simulink model "hdlcordic_eml"  (R2026a)
settings: Solver=FixedStepDiscrete  StopTime=720
InitFcn:
  | rate = 8;
libraries: simulink_need_slupdate x2, simulink x1
Description:
  | CORDIC Algorithm Using the MATLAB(R) Function Block
  | This example shows how to use HDL Coder(TM) to check, generate and
  | verify HDL for a fixed-point CORDIC model implementing sin and cos
  | trigonometric functions using the MATLAB Function Block.
settings Model: Creator=The MathWorks, Inc.  LastModifiedBy=The MathWorks, Inc.
settings OptimizationCC: ConditionallyExecuteInputs=off  InitFltsAndDblsToZero=on  EfficientMapNaN2IntZero=off
settings DebuggingCC: SaveWithParameterizedLinksMsg=none  UnderspecifiedInitializationDetection=Classic  SingleTaskRateTransMsg=error  IntegerOverflowMsg=none  ParameterDowncastMsg=none  ParameterOverflowMsg=none  ParameterPrecisionLossMsg=none  ParameterTunabilityLossMsg=none  IntegerSaturationMsg=none
settings HardwareCC: ProdHWDeviceType=ASIC/FPGA  TargetHWDeviceType=32-bit Generic  ProdEqTarget=off
settings GRTTargetCC: TargetFcnLib=ansi_tfl_tmw_new.mat  CombineOutputUpdateFcns=off  GRTInterface=on

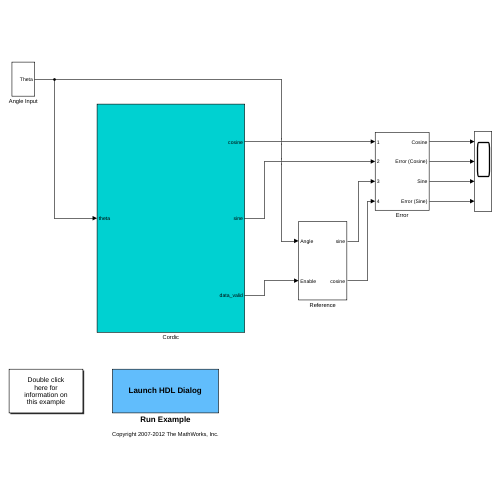
[thumbnail: Simulink's stored preview of the top-level diagram]
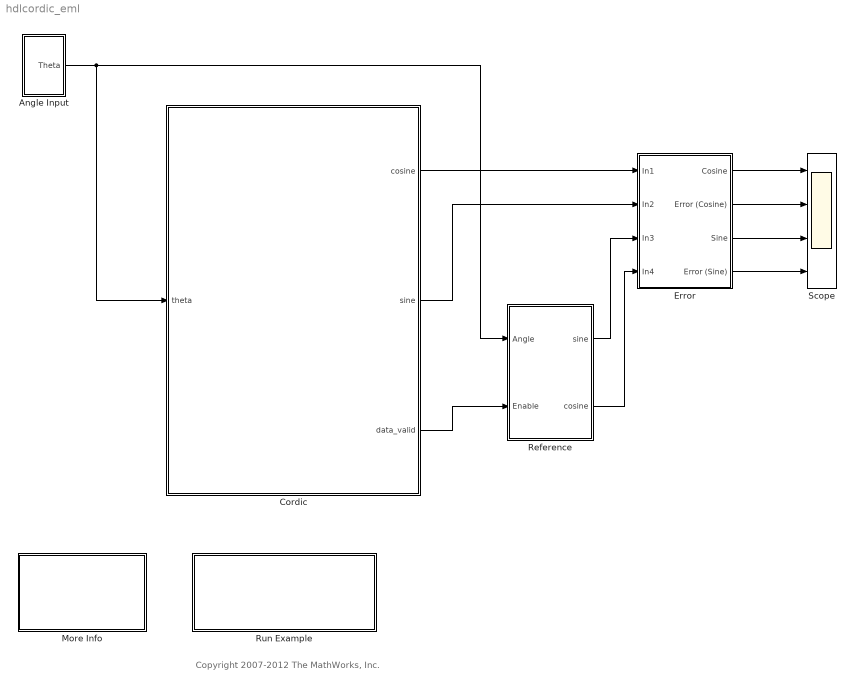
== system hdlcordic_eml ==
  note: Copyright 2007-2012 The MathWorks, Inc.
  Angle Input : Subsystem
  Cordic : Subsystem
  Error : Subsystem
  More Info : Subsystem
      mask Display: disp('Double click\nhere for\ninformation on\nthis example')
  Reference : Subsystem
  Run Example : Subsystem
      settings: OpenFcn=hdldialog(bdroot)
      mask Display: disp('Launch HDL Dialog')
  Scope : Scope  NumInputPorts=4
      settings: TimeSpan=800  Title=Cosine_Reference (Yellow) vs Cosine_Cordic (Purple)  ActiveDisplayYMinimum=-1  ActiveDisplayYMaximum=1
  wires:
  Angle Input/1(Theta) -> Reference/1(Angle), Cordic/1(theta)
  Reference/1(sine) -> Error/3(In3)
  Reference/2(cosine) -> Error/4(In4)
  Error/1(Cosine) -> Scope/1
  Error/2(Error (Cosine)) -> Scope/2
  Error/3(Sine) -> Scope/3
  Error/4(Error (Sine)) -> Scope/4
  Cordic/1(cosine) -> Error/1(In1)
  Cordic/2(sine) -> Error/2(In2)
  Cordic/3(data_valid) -> Reference/2(Enable)

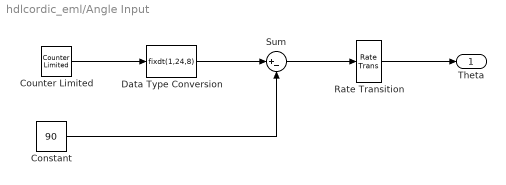
== system hdlcordic_eml/Angle Input ==
  Constant : Constant  Value=90  OutDataTypeStr=fixdt(1,24,8)  SampleTime=1
  Counter Limited : simulink/Sources/Counter Limited  uplimit=360  tsamp=1
  Data Type Conversion : DataTypeConversion  OutDataTypeStr=fixdt(1,24,8)  SaturateOnIntegerOverflow=off  RndMeth=Floor
  Rate Transition : RateTransition  OutPortSampleTime=1/rate
  Sum : Sum  Inputs=|+-  OutDataTypeStr=fixdt(1, 24, 8)
  Theta : Outport
  wires:
  Rate Transition/1 -> Theta/1
  Sum/1 -> Rate Transition/1
  Data Type Conversion/1 -> Sum/1
  Constant/1 -> Sum/2
  Counter Limited/1 -> Data Type Conversion/1

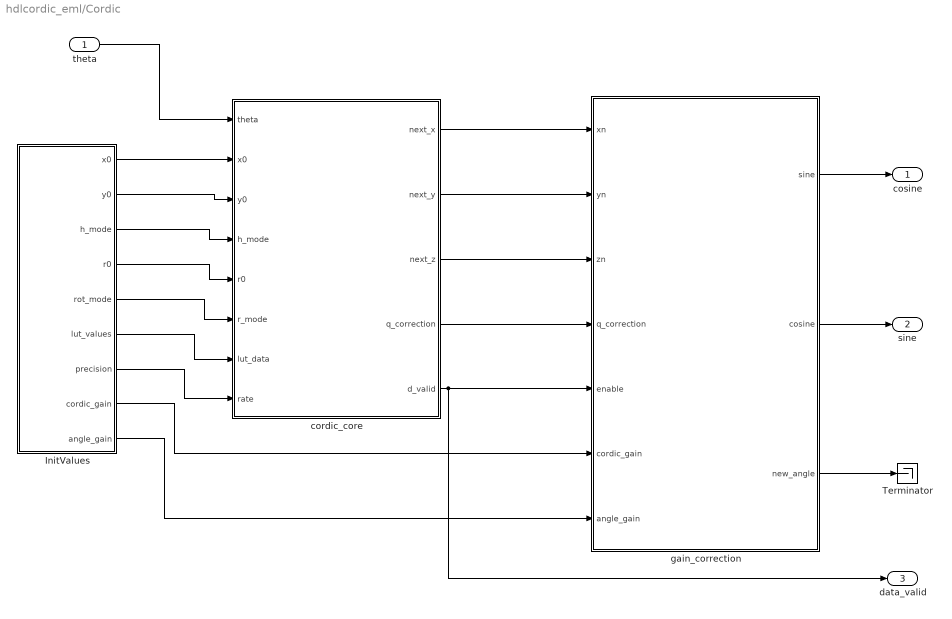
== system hdlcordic_eml/Cordic ==
  theta : Inport
  InitValues : Subsystem
  Terminator : Terminator
  cordic_core : Subsystem
  gain_correction : MATLAB Function  TreatAsAtomicUnit=on
  cosine : Outport
  sine : Outport  Port=2
  data_valid : Outport  Port=3
  wires:
  gain_correction/1(sine) -> cosine/1
  gain_correction/2(cosine) -> sine/1
  gain_correction/3(new_angle) -> Terminator/1
  cordic_core/1(next_x) -> gain_correction/1(xn)
  cordic_core/2(next_y) -> gain_correction/2(yn)
  cordic_core/3(next_z) -> gain_correction/3(zn)
  cordic_core/4(q_correction) -> gain_correction/4(q_correction)
  cordic_core/5(d_valid) -> gain_correction/5(enable), data_valid/1
  InitValues/8(cordic_gain) -> gain_correction/6(cordic_gain)
  InitValues/9(angle_gain) -> gain_correction/7(angle_gain)
  theta/1 -> cordic_core/1(theta)
  InitValues/1(x0) -> cordic_core/2(x0)
  InitValues/2(y0) -> cordic_core/3(y0)
  InitValues/3(h_mode) -> cordic_core/4(h_mode)
  InitValues/4(r0) -> cordic_core/5(r0)
  InitValues/5(rot_mode) -> cordic_core/6(r_mode)
  InitValues/6(lut_values) -> cordic_core/7(lut_data)
  InitValues/7(precision) -> cordic_core/8(rate)

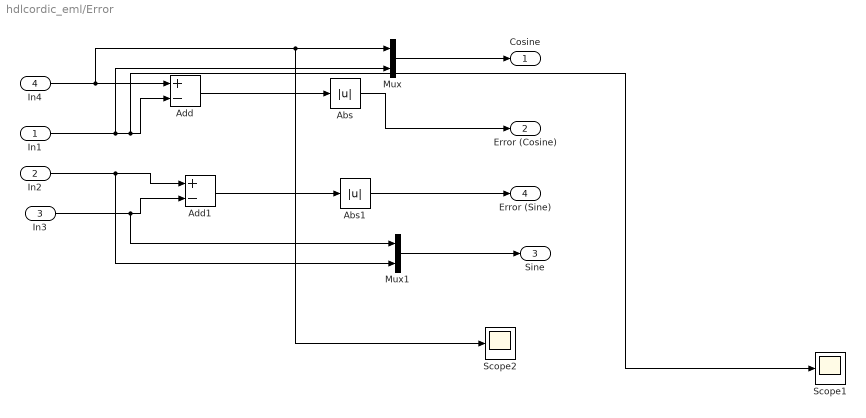
== system hdlcordic_eml/Error ==
  In1 : Inport
  In2 : Inport  Port=2
  In3 : Inport  Port=3
  In4 : Inport  Port=4
  Abs : Abs  SaturateOnIntegerOverflow=off
  Abs1 : Abs  SaturateOnIntegerOverflow=off
  Add : Sum  Inputs=+-  OutDataTypeStr=Inherit: Inherit via back propagation
  Add1 : Sum  Inputs=+-  OutDataTypeStr=Inherit: Inherit via back propagation
  Mux : Mux  Inputs=2
  Mux1 : Mux  Inputs=2
  Scope1 : Scope
      settings: ActiveDisplayYMinimum=0.7125  ActiveDisplayYMaximum=0.7875  DataLoggingVariableName=ScopeData3
  Scope2 : Scope
      settings: ActiveDisplayYMinimum=0.1  ActiveDisplayYMaximum=0.8  DataLoggingVariableName=ScopeData2
  Cosine : Outport
  Error (Cosine) : Outport  Port=2
  Sine : Outport  Port=3
  Error (Sine) : Outport  Port=4
  wires:
  In4/1 -> Add/1, Mux/1, Scope2/1
  In1/1 -> Mux/2, Add/2, Scope1/1
  In2/1 -> Add1/1, Mux1/2
  In3/1 -> Add1/2, Mux1/1
  Add1/1 -> Abs1/1
  Add/1 -> Abs/1
  Abs/1 -> Error (Cosine)/1
  Mux/1 -> Cosine/1
  Abs1/1 -> Error (Sine)/1
  Mux1/1 -> Sine/1

== system hdlcordic_eml/More Info ==
  note: MATLAB Function Block CORDIC Example
  note: This example shows how to implement the CORDIC algorithm solely using
      | MATLAB Function blocks.
      |
      | CORDIC is a shift-add based algorithm suitable for HDL code generation.
      | For complete details see the following reference paper.
      |
      | A survey of CORDIC algorithms for FPGAs
      | Ray Andraka, FPGA '98. Proceedings of the
      | 1998 ACM/SIGDA sixth international symposium on Field programmable gate arrays,
      | Feb. 22-24, 1998, Monterey, CA. pp191-200.
  note: For Verilog:
      |
      |   makehdl('hdlcordic_eml/Cordic', 'TargetLanguage', 'Verilog')
      |   makehdltb('hdlcordic_eml/Cordic', 'TargetLanguage', 'Verilog')
      |
      | For VHDL:
      |
      |   makehdl('hdlcordic_eml/Cordic', 'TargetLanguage', 'Vhdl')
      |   makehdltb('hdlcordic_eml/Cordic', 'TargetLanguage', 'Vhdl')
  note: In MATLAB(R), type the following:

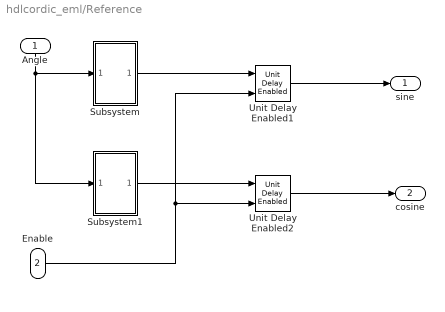
== system hdlcordic_eml/Reference ==
  Angle : Inport
  Enable : Inport  Port=2
  Subsystem : Subsystem
      mask Display: disp('Sine')
  Subsystem1 : Subsystem
      mask Display: disp('Cosine')
  Unit Delay Enabled1 : simulink_need_slupdate/Unit Delay Enabled  vinit=0  tsamp=1/rate
  Unit Delay Enabled2 : simulink_need_slupdate/Unit Delay Enabled  vinit=0  tsamp=1/rate
  sine : Outport
  cosine : Outport  Port=2
  wires:
  Angle/1 -> Subsystem/1(In1), Subsystem1/1(In1)
  Subsystem/1(Out1) -> Unit Delay Enabled1/1
  Unit Delay Enabled1/1 -> sine/1
  Enable/1 -> Unit Delay Enabled1/2, Unit Delay Enabled2/2
  Subsystem1/1(Out1) -> Unit Delay Enabled2/1
  Unit Delay Enabled2/1 -> cosine/1

== system hdlcordic_eml/Run Example ==

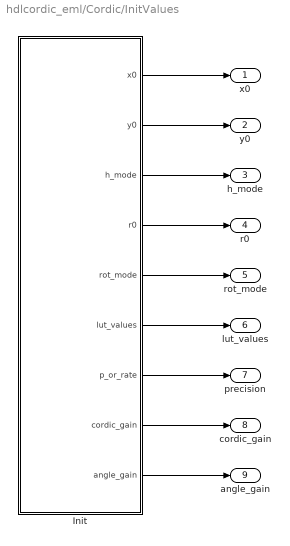
== system hdlcordic_eml/Cordic/InitValues ==
  Init : MATLAB Function  TreatAsAtomicUnit=on
  x0 : Outport
  y0 : Outport  Port=2
  h_mode : Outport  Port=3
  r0 : Outport  Port=4
  rot_mode : Outport  Port=5
  lut_values : Outport  Port=6
  precision : Outport  Port=7
  cordic_gain : Outport  Port=8
  angle_gain : Outport  Port=9
  wires:
  Init/1(x0) -> x0/1
  Init/2(y0) -> y0/1
  Init/3(h_mode) -> h_mode/1
  Init/4(r0) -> r0/1
  Init/5(rot_mode) -> rot_mode/1
  Init/6(lut_values) -> lut_values/1
  Init/7(p_or_rate) -> precision/1
  Init/8(cordic_gain) -> cordic_gain/1
  Init/9(angle_gain) -> angle_gain/1

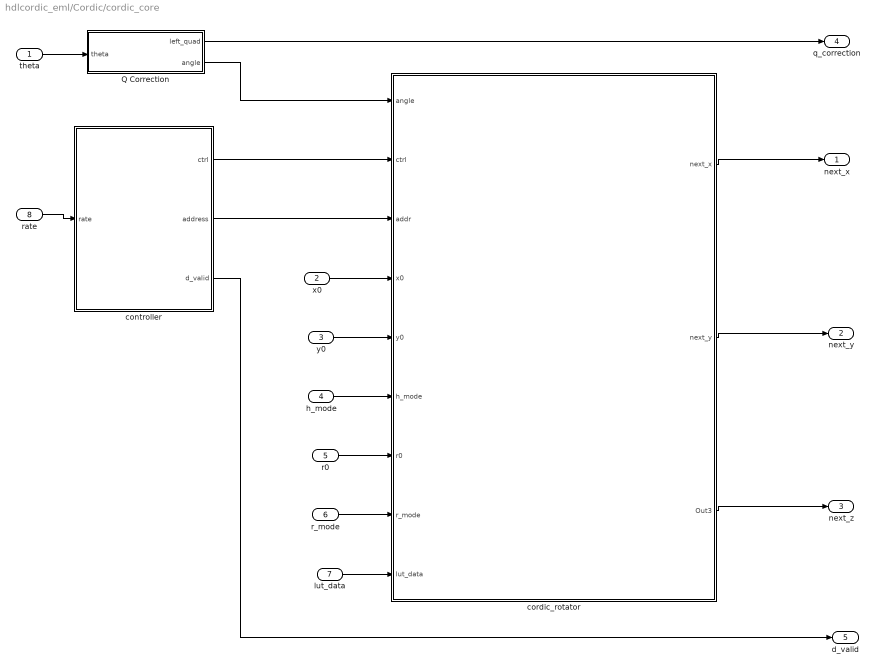
== system hdlcordic_eml/Cordic/cordic_core ==
  theta : Inport
  x0 : Inport  Port=2
  y0 : Inport  Port=3
  h_mode : Inport  Port=4
  r0 : Inport  Port=5
  r_mode : Inport  Port=6
  lut_data : Inport  Port=7
  rate : Inport  Port=8
  Q Correction : MATLAB Function  TreatAsAtomicUnit=on
  controller : MATLAB Function  TreatAsAtomicUnit=on
  cordic_rotator : Subsystem
  next_x : Outport
  next_y : Outport  Port=2
  next_z : Outport  Port=3
  q_correction : Outport  Port=4
  d_valid : Outport  Port=5
  wires:
  controller/3(d_valid) -> d_valid/1
  rate/1 -> controller/1(rate)
  cordic_rotator/2(next_y) -> next_y/1
  cordic_rotator/1(next_x) -> next_x/1
  cordic_rotator/3(Out3) -> next_z/1
  theta/1 -> Q Correction/1(theta)
  Q Correction/1(left_quad) -> q_correction/1
  x0/1 -> cordic_rotator/4(x0)
  h_mode/1 -> cordic_rotator/6(h_mode)
  r0/1 -> cordic_rotator/7(r0)
  r_mode/1 -> cordic_rotator/8(r_mode)
  lut_data/1 -> cordic_rotator/9(lut_data)
  y0/1 -> cordic_rotator/5(y0)
  Q Correction/2(angle) -> cordic_rotator/1(angle)
  controller/1(ctrl) -> cordic_rotator/2(ctrl)
  controller/2(address) -> cordic_rotator/3(addr)

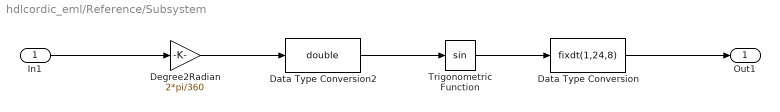
== system hdlcordic_eml/Reference/Subsystem ==
  In1 : Inport
  Data Type Conversion : DataTypeConversion  OutDataTypeStr=fixdt(1,24,8)  SaturateOnIntegerOverflow=off  RndMeth=Floor
  Data Type Conversion2 : DataTypeConversion  OutDataTypeStr=double  SaturateOnIntegerOverflow=off  RndMeth=Floor
  Degree2Radian : Gain  Gain=2*pi/360  OutDataTypeStr=Inherit: Same as input
  Trigonometric Function : Trigonometry
  Out1 : Outport
  wires:
  Trigonometric Function/1 -> Data Type Conversion/1
  Data Type Conversion/1 -> Out1/1
  In1/1 -> Degree2Radian/1
  Data Type Conversion2/1 -> Trigonometric Function/1
  Degree2Radian/1 -> Data Type Conversion2/1

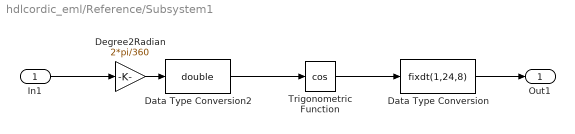
== system hdlcordic_eml/Reference/Subsystem1 ==
  In1 : Inport
  Data Type Conversion : DataTypeConversion  OutDataTypeStr=fixdt(1,24,8)  SaturateOnIntegerOverflow=off  RndMeth=Floor
  Data Type Conversion2 : DataTypeConversion  OutDataTypeStr=double  SaturateOnIntegerOverflow=off  RndMeth=Floor
  Degree2Radian : Gain  Gain=2*pi/360
  Trigonometric Function : Trigonometry  Operator=cos
  Out1 : Outport
  wires:
  Data Type Conversion/1 -> Out1/1
  Degree2Radian/1 -> Data Type Conversion2/1
  Trigonometric Function/1 -> Data Type Conversion/1
  Data Type Conversion2/1 -> Trigonometric Function/1
  In1/1 -> Degree2Radian/1

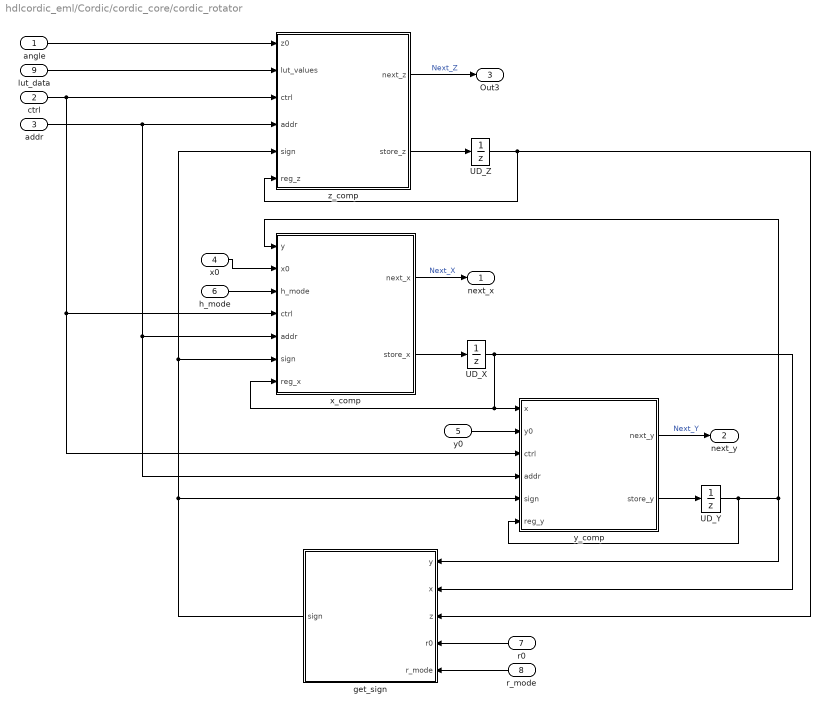
== system hdlcordic_eml/Cordic/cordic_core/cordic_rotator ==
  angle : Inport
  ctrl : Inport  Port=2
  addr : Inport  Port=3
  x0 : Inport  Port=4
  y0 : Inport  Port=5
  h_mode : Inport  Port=6
  r0 : Inport  Port=7
  r_mode : Inport  Port=8
  lut_data : Inport  Port=9
  UD_X : UnitDelay  SampleTime=-1
  UD_Y : UnitDelay  SampleTime=-1
  UD_Z : UnitDelay  SampleTime=-1
  get_sign : MATLAB Function  TreatAsAtomicUnit=on
  x_comp : MATLAB Function  TreatAsAtomicUnit=on
  y_comp : MATLAB Function  TreatAsAtomicUnit=on
  z_comp : MATLAB Function  TreatAsAtomicUnit=on
  next_x : Outport
  next_y : Outport  Port=2
  Out3 : Outport  Port=3
  wires:
  r_mode/1 -> get_sign/5(r_mode)
  r0/1 -> get_sign/4(r0)
  addr/1 -> y_comp/4(addr), x_comp/5(addr), z_comp/4(addr)
  ctrl/1 -> y_comp/3(ctrl), x_comp/4(ctrl), z_comp/3(ctrl)
  lut_data/1 -> z_comp/2(lut_values)
  y0/1 -> y_comp/2(y0)
  h_mode/1 -> x_comp/3(h_mode)
  x0/1 -> x_comp/2(x0)
  y_comp/2(store_y) -> UD_Y/1
  get_sign/1(sign) -> y_comp/5(sign), z_comp/5(sign), x_comp/6(sign)
  UD_Z/1 -> z_comp/6(reg_z), get_sign/3(z)
  UD_Y/1 -> y_comp/6(reg_y), get_sign/1(y), x_comp/1(y)
  UD_X/1 -> y_comp/1(x), x_comp/7(reg_x), get_sign/2(x)
  x_comp/2(store_x) -> UD_X/1
  z_comp/2(store_z) -> UD_Z/1
  angle/1 -> z_comp/1(z0)
  x_comp/1(next_x) -> next_x/1  "Next_X"
  y_comp/1(next_y) -> next_y/1  "Next_Y"
  z_comp/1(next_z) -> Out3/1  "Next_Z"

== matlab function hdlcordic_eml/Cordic/InitValues/Init ==
  settings: fimath=|
      | fimath(...
      | 'RoundMode', 'floor',...
      | 'OverflowMode', 'wrap',...
      | 'ProductMode', 'FullPrecision', 'ProductWordLength', 32,...
      | 'SumMode', 'FullPrecision', 'SumWordLength', 32,...
      | 'CastBeforeSum', true)
  data: x0 output fixdt(1,24,8); y0 output fixdt(1,24,8); h_mode output boolean; r0 output fixdt(1,24,8); rot_mode output uint8; lut_values output fixdt(1,16,8) size=[1 8]; p_or_rate output uint8; cordic_gain output fixdt(1,24,23); angle_gain output fixdt(1,24,22)
function [x0, y0, ...    
    h_mode,...
    r0, rot_mode, ...    
    lut_values, ...
    p_or_rate, ...
    cordic_gain, ...
    angle_gain] = INIT


rate = 8;

% from mask input
p_or_rate = uint8(rate);

x0 = getfi(1); 
y0 = getfi(0);

r0 = getfi(0);

% hyperbolic mode
h_mode = false;

% rotation mode
rot_mode = uint8(2); 

%cg = 1/get_cordic_gain(8, 'Circular');
%cordic_gain = fi(cg, 1, 24, 23);
cordic_gain = fi(0.607259154319763, 1, 24, 23);

angle_gain = fi(1, 1, 24, 22);

%sincos_val = (atan([1, 1/2, 1/4, 1/8, 1/16, 1/32, 1/64, 1/128]))*180/pi;
%lut_values = fi(sincos_val, 1, 16, 8);

lut_values = fi([45, 26.56640625, 14.03515625, 7.125, 3.578125, 1.7890625, 0.89453125, 0.44921875], 1, 16, 8);


function fival = getfi(val)
coder.inline('always');

nt = numerictype(1, 24, 8);

fm = fimath(...
    'RoundMode', 'floor',...
    'OverflowMode', 'wrap',...
    'ProductMode', 'FullPrecision', 'ProductWordLength', 32,...
    'SumMode', 'FullPrecision', 'SumWordLength', 32,...
    'CastBeforeSum', true);

fival = fi(val, nt, fm);

== matlab function hdlcordic_eml/Cordic/gain_correction ==
  settings: updateMethod=DISCRETE  sampleTime=1/rate
  settings: fimath=|
      | fimath(...
      | 'RoundMode', 'floor',...
      | 'OverflowMode', 'wrap',...
      | 'ProductMode', 'SpecifyPrecision', 'ProductWordLength', 32,...
      | 'SumMode', 'SpecifyPrecision', 'SumWordLength', 32,...
      | 'CastBeforeSum', true)
  data: sine output fixdt(1,24,8); cosine output fixdt(1,24,8); xn input fixdt(1,24,8); yn input fixdt(1,24,8); zn input fixdt(1,24,8); q_correction input boolean; enable input boolean; cordic_gain input fixdt(1,24,23); angle_gain input fixdt(1,24,22); new_angle output fixdt(1,24,8)
function [sine, cosine, new_angle] = gain_correction(xn, yn, zn, q_correction, enable, cordic_gain, angle_gain)

persistent x_reg;
if isempty(x_reg)
    x_reg = getfi(0);
end

persistent y_reg;
if isempty(y_reg)
    y_reg = getfi(0);
end

persistent z_reg;
if isempty(z_reg)
    z_reg = getfi(0);
end

xg = getfi(cordic_gain*xn);
yg = getfi(cordic_gain*yn);

[xout, yout] = vector_correction(xg, yg, cordic_gain, q_correction);
zout = z_correction(zn, q_correction, angle_gain);

sine = x_reg;
cosine = y_reg;
new_angle = z_reg;

if (enable)
    x_reg = xout;
    y_reg = yout;
    z_reg = zout;
end

function [xout, yout] = vector_correction(x, y, c0, q_correction)

if q_correction
    direction = getfi(-1);
else
    direction = getfi(1);
end

xout = getfi(x*direction);
yout = getfi(y*direction);


function z_c = z_correction(zn, z_corr, z_gain)

t1 = getfi(zn);
t2 = getfi(uint8(z_corr));
zadd = getfi(t1+t2);

z_c = getfi(zadd * z_gain);



function fival = getfi(val)

nt = numerictype(1, 24, 8);

fm = fimath(...
    'RoundMode', 'floor',...
    'OverflowMode', 'wrap',...
    'ProductMode', 'SpecifyPrecision', 'ProductWordLength', 32,...
    'SumMode', 'SpecifyPrecision', 'SumWordLength', 32,...
    'CastBeforeSum', true);

fival = fi(val, nt, fm);

== matlab function hdlcordic_eml/Cordic/cordic_core/Q Correction ==
  settings: fimath=|
      | fimath(...
      | 'RoundMode', 'floor',...
      | 'OverflowMode', 'wrap',...
      | 'ProductMode', 'FullPrecision', 'ProductWordLength', 32,...
      | 'SumMode', 'FullPrecision', 'SumWordLength', 32,...
      | 'CastBeforeSum', true)
  data: theta input; left_quad output; angle output
function [left_quad, angle] = Q_Correction(theta)

angle = theta;
left_quad = angle <= 270 && angle >= 90;

if left_quad
    angle = getfi(angle - getfi(180));
end


function fival = getfi(val)

nt = numerictype(1, 24, 8);

fm = fimath(...
    'RoundMode', 'floor',...
    'OverflowMode', 'wrap',...
    'ProductMode', 'FullPrecision', 'ProductWordLength', 32,...
    'SumMode', 'FullPrecision', 'SumWordLength', 32,...
    'CastBeforeSum', true);

fival = fi(val, nt, fm);

== matlab function hdlcordic_eml/Cordic/cordic_core/controller ==
  settings: updateMethod=DISCRETE  sampleTime=1/rate
  settings: fimath=|
      | fimath(...
      | 'RoundMode', 'floor',...
      | 'OverflowMode', 'wrap',...
      | 'ProductMode', 'FullPrecision', 'ProductWordLength', 32,...
      | 'SumMode', 'FullPrecision', 'SumWordLength', 32,...
      | 'CastBeforeSum', true)
  data: ctrl output; address output; d_valid output; rate input
function [ctrl,address,d_valid] = controller(rate)

persistent count;
if isempty(count)
    count = uint8(1);
end

% output address
address = count;

% update count value
count = get_en_ctr_val(rate);

% send control signals based on current count value
ctrl = (count == 1);
d_valid = (count == 8);



function count = get_en_ctr_val(rate)

persistent count_val;
if isempty(count_val)
    count_val = uint8(1);
end

% output count
count = count_val;

% update count
if count >= rate
    next_cnt_val = uint8(1);
else
    next_cnt_val = uint8(count+1);
end


count_val = uint8(next_cnt_val);

== matlab function hdlcordic_eml/Cordic/cordic_core/cordic_rotator/get_sign ==
  settings: fimath=|
      | fimath(...
      | 'RoundMode', 'floor',...
      | 'OverflowMode', 'wrap',...
      | 'ProductMode', 'FullPrecision', 'ProductWordLength', 32,...
      | 'SumMode', 'FullPrecision', 'SumWordLength', 32,...
      | 'CastBeforeSum', true)
  data: y input; x input; z input; r0 input; sign output boolean; r_mode input
function sign = get_sign(y, x, z, r0, r_mode)

sign = false;

switch (r_mode)
    case 0
        sign = x <= r0;
    case 1
        sign = y  <= r0;
    case 2
        sign = z >= r0;
end

== matlab function hdlcordic_eml/Cordic/cordic_core/cordic_rotator/x_comp ==
  settings: fimath=|
      | fimath(...
      | 'RoundMode', 'floor',...
      | 'OverflowMode', 'wrap',...
      | 'ProductMode', 'FullPrecision', 'ProductWordLength', 32,...
      | 'SumMode', 'FullPrecision', 'SumWordLength', 32,...
      | 'CastBeforeSum', true)
  data: y input fixdt(1,24,8) size=1; next_x output fixdt(1,24,8) size=1; x0 input fixdt(1,24,8) size=1; h_mode input boolean size=1; ctrl input boolean size=1; addr input uint8 size=1; sign input boolean; store_x output fixdt(1,24,8); reg_x input fixdt(1,24,8)
function [next_x, store_x]   = x_comp(y, x0, h_mode, ctrl, addr, sign, reg_x)

y = bitshift(y, -int8(addr-1));

if h_mode    
    new_sign = sign;
else
    new_sign = ~sign;
end

next_x = z_accumulator(new_sign, reg_x, y);

% update delay line
if (ctrl)
    store_x = x0;
else
    store_x = next_x;
end


function acc = z_accumulator(add, x, y)

if (add)
    acc = getfi(x+y);
else
    acc = getfi(x-y);
end


function fival = getfi(val)

nt = numerictype(1, 24, 8);
fm = fimath(...
    'RoundMode', 'floor',...
    'OverflowMode', 'wrap',...
    'ProductMode', 'FullPrecision', 'ProductWordLength', 32,...
    'SumMode', 'FullPrecision', 'SumWordLength', 32,...
    'CastBeforeSum', true);

fival = fi(val, nt, fm);

== matlab function hdlcordic_eml/Cordic/cordic_core/cordic_rotator/y_comp ==
  settings: fimath=|
      | fimath(...
      | 'RoundMode', 'floor',...
      | 'OverflowMode', 'wrap',...
      | 'ProductMode', 'FullPrecision', 'ProductWordLength', 32,...
      | 'SumMode', 'FullPrecision', 'SumWordLength', 32,...
      | 'CastBeforeSum', true)
  data: next_y output fixdt(1,24,8); x input fixdt(1,24,8); y0 input fixdt(1,24,8); ctrl input boolean; addr input uint8; sign input boolean; store_y output fixdt(1,24,8); reg_y input fixdt(1,24,8)
function [next_y, store_y]  = y_comp(x, y0, ctrl, addr, sign, reg_y)

x = bitshift(x, -int8(addr-1));

next_y = z_accumulator(sign, x, reg_y);

if (ctrl)
    store_y = y0;
else
    store_y = next_y;
end


function acc = z_accumulator(add, x, y)

if (add)
    acc = getfi(y+x);
else
    acc = getfi(y-x);
end

function fival = getfi(val)

nt = numerictype(1, 24, 8);

fm = fimath(...
    'RoundMode', 'floor',...
    'OverflowMode', 'wrap',...
    'ProductMode', 'FullPrecision', 'ProductWordLength', 32,...
    'SumMode', 'FullPrecision', 'SumWordLength', 32,...
    'CastBeforeSum', true);

fival = fi(val, nt, fm);

== matlab function hdlcordic_eml/Cordic/cordic_core/cordic_rotator/z_comp ==
  settings: fimath=|
      | fimath(...
      | 'RoundMode', 'floor',...
      | 'OverflowMode', 'wrap',...
      | 'ProductMode', 'FullPrecision', 'ProductWordLength', 32,...
      | 'SumMode', 'FullPrecision', 'SumWordLength', 32,...
      | 'CastBeforeSum', true)
  data: next_z output fixdt(1,24,8); z0 input fixdt(1,24,8); lut_values input fixdt(1,16,8) size=[1 8]; ctrl input boolean; addr input uint8; sign input boolean; reg_z input fixdt(1,24,8); store_z output
function [next_z, store_z]   = z_comp(z0, lut_values, ctrl, addr, sign, reg_z)

y = lut_values(addr);

%sign = ~sign;
next_z = z_accumulator(~sign, reg_z, y);

% update delay line
if (ctrl)
    store_z = z0;
else
    store_z = next_z;
end

function acc = z_accumulator(add, x, y)

if (add)
    acc = getfi(x+y);
else
    acc = getfi(x-y);
end


function fival = getfi(val)

nt = numerictype(1, 24, 8);

fm = fimath(...
    'RoundMode', 'floor',...
    'OverflowMode', 'wrap',...
    'ProductMode', 'FullPrecision', 'ProductWordLength', 32,...
    'SumMode', 'FullPrecision', 'SumWordLength', 32,...
    'CastBeforeSum', true);

fival = fi(val, nt, fm);
